simulink model "AFC_FFNN_trainscg_15_15_15_15_15_ctr_Nor_July_15"  (R2021a)
settings: Solver=VariableStepAuto  StartTime=0.0  StopTime=10.0  RelTol=1e-3
libraries: neural x82
(part 3 of 3)

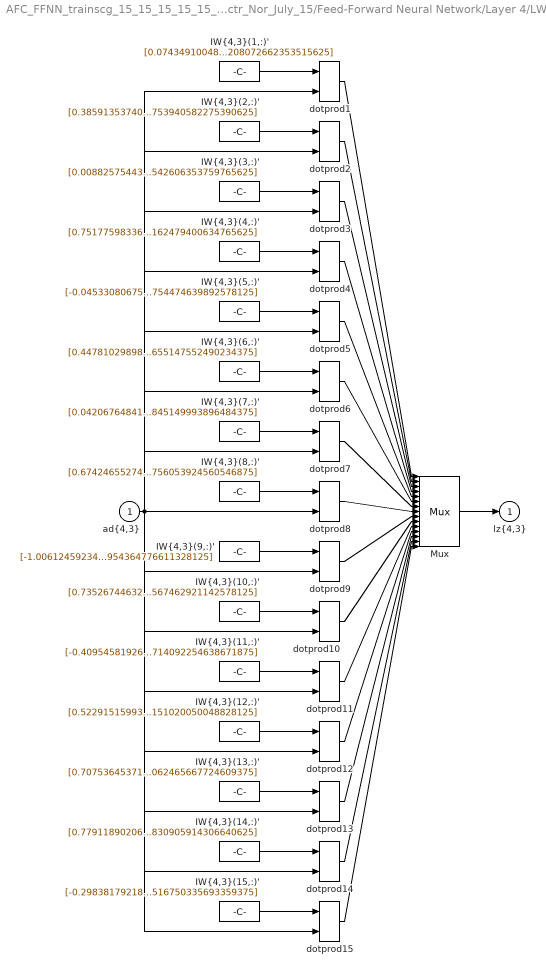
== system AFC_FFNN_trainscg_15_15_15_15_15_ctr_Nor_July_15/Feed-Forward Neural Network/Layer 4/LW{4,3} ==
  "ad{4,3}" : Inport  PortDimensions=15
      mask Display: e = 0.06;c1 = [120 230 180]/255;c2 = ([120 230 180]+0)/(256+128);c3 = ([120 230 180]+128)/(256+128);patch([0 1 1 0],[0 0 1 1],c1);patch([0 1 1 1-e 1-e 0+e],[0 0 1 1-e 0+e 0+e],c2);patch([0 0 1 1-e 0+e 0+e],[0 1 1 1-e 1-e 0+e],c3);plot([0 1 1 0 0],[0 0 1 1 0]);
  "IW{4,3}(1,:)'" : Constant  Value=[0.074349100483344032763710629296838305890560150146484375;-0.2325662791511675653310931011219508945941925048828125;-0.5381154884542291849669481962337158620357513427734375;0.1386295109502034550441607052562176249921321868896484375;-0.37797625642184240479792833866667933762073516845703125;0.6500953139118197388057751595624722540378570556640625;-0.71645051950191429579462010224233381450176239013671875;-0.42415904949149141334174828443792648613452911376953125;-0.522087717682781171646411166875623166561126708984375;0.2134427609428042327266439315280877053737640380859375;-0.9265960947882854181756329126073978841304779052734375;-0.1461549422446244417272964710718952119350433349609375;0.496156728707464911298785636972752399742603302001953125;-0.467980089049811087686947530528414063155651092529296875;-0.828161988219234590502537685097195208072662353515625]
      mask Display: e = 0.06;c1 = [120 150 230]/255;c2 = ([120 150 230]+0)/383;c3 = ([120 150 230]+128)/383;patch([0 1 1 0],[0 0 1 1],c1);patch([0 1 1 1-e 1-e 0+e],[0 0 1 1-e 0+e 0+e],c2);patch([0 0 1 1-e 0+e 0+e],[0 1 1 1-e 1-e 0+e],c3);plot([0 1 1 0 0],[0 0 1 1 0]);disp('weights');
  "IW{4,3}(10,:)'" : Constant  Value=[0.7352674463222312883914355552406050264835357666015625;-0.6220688627615544863402874398161657154560089111328125;-0.4612868378094046040160947086405940353870391845703125;-0.7690744341636996939115533677977509796619415283203125;0.364523315808154446671096593490801751613616943359375;-0.5505544008294369628941922201192937791347503662109375;0.9440421013235733571633545579970814287662506103515625;-0.2344205461328694450884313482674770057201385498046875;-0.3421493061719094175288091719266958534717559814453125;-0.7250516891389173768089904115186072885990142822265625;-0.2911601662961176284483144627301953732967376708984375;0.4865548552326515174826226939330808818340301513671875;-0.614256005760669854254274468985386192798614501953125;-0.14911166211352355759345300612039864063262939453125;0.9353193529802219519098116506938822567462921142578125]
      mask Display: e = 0.06;c1 = [120 150 230]/255;c2 = ([120 150 230]+0)/383;c3 = ([120 150 230]+128)/383;patch([0 1 1 0],[0 0 1 1],c1);patch([0 1 1 1-e 1-e 0+e],[0 0 1 1-e 0+e 0+e],c2);patch([0 0 1 1-e 0+e 0+e],[0 1 1 1-e 1-e 0+e],c3);plot([0 1 1 0 0],[0 0 1 1 0]);disp('weights');
  "IW{4,3}(11,:)'" : Constant  Value=[-0.40954581926718258699793295818381011486053466796875;-0.209952151050021740275042247958481311798095703125;-0.2064904433647580805910592971486039459705352783203125;0.1238876984131753733464620381710119545459747314453125;0.2207973745056917014295549961389042437076568603515625;0.4043229885403072376703903501038439571857452392578125;0.16052297693793082800084448535926640033721923828125;-0.1510627772562316284421513046254403889179229736328125;0.625340446388026105495328010874800384044647216796875;-0.737940333490474387190261040814220905303955078125;-0.081506414055812381747045947122387588024139404296875;0.5640702366617400542736504576168954372406005859375;-0.1445523819865301984322059070109389722347259521484375;-0.573360915257262515609681940986774861812591552734375;0.36503182909853659765531119774095714092254638671875]
      mask Display: e = 0.06;c1 = [120 150 230]/255;c2 = ([120 150 230]+0)/383;c3 = ([120 150 230]+128)/383;patch([0 1 1 0],[0 0 1 1],c1);patch([0 1 1 1-e 1-e 0+e],[0 0 1 1-e 0+e 0+e],c2);patch([0 0 1 1-e 0+e 0+e],[0 1 1 1-e 1-e 0+e],c3);plot([0 1 1 0 0],[0 0 1 1 0]);disp('weights');
  "IW{4,3}(12,:)'" : Constant  Value=[0.5229151599398147443054085670155473053455352783203125;0.0668062429593738738020647360826842486858367919921875;0.10388454329580172619262867783618276007473468780517578125;-0.6445508987129973110796754554030485451221466064453125;0.10760557398696679598515402176417410373687744140625;-0.8975738027855137968202825504704378545284271240234375;0.4048106195281306884936611822922714054584503173828125;0.7646290355386236026191681958152912557125091552734375;0.808722577754244387193693910376168787479400634765625;-0.369588474634115815575796659686602652072906494140625;0.927177911226604312133758867275901138782501220703125;0.2464285148358735799689611667417921125888824462890625;-0.7710168032929891612781148069188930094242095947265625;0.9789119736813682859377649947418831288814544677734375;-0.4766114794815010657913489922066219151020050048828125]
      mask Display: e = 0.06;c1 = [120 150 230]/255;c2 = ([120 150 230]+0)/383;c3 = ([120 150 230]+128)/383;patch([0 1 1 0],[0 0 1 1],c1);patch([0 1 1 1-e 1-e 0+e],[0 0 1 1-e 0+e 0+e],c2);patch([0 0 1 1-e 0+e 0+e],[0 1 1 1-e 1-e 0+e],c3);plot([0 1 1 0 0],[0 0 1 1 0]);disp('weights');
  "IW{4,3}(13,:)'" : Constant  Value=[0.7075364537119337438042521171155385673046112060546875;-0.767668879818697913464120574644766747951507568359375;0.55007147010354884297811395299504511058330535888671875;-0.6106701140328276711244370744680054485797882080078125;0.6972476042524231587549365940503776073455810546875;-0.5354868194475292941802990753785707056522369384765625;0.76167148072680157522285071536316536366939544677734375;-0.42180889329320836456105325851240195333957672119140625;0.7665122361950833518307035774341784417629241943359375;0.90348869713702295580759482618304900825023651123046875;-0.07351895802781971411832273588515818119049072265625;-0.32664730128458874247598942019976675510406494140625;0.6420791870935589340518845347105525434017181396484375;0.74761179512886855036413180641829967498779296875;0.0630118524273972635540985720581375062465667724609375]
      mask Display: e = 0.06;c1 = [120 150 230]/255;c2 = ([120 150 230]+0)/383;c3 = ([120 150 230]+128)/383;patch([0 1 1 0],[0 0 1 1],c1);patch([0 1 1 1-e 1-e 0+e],[0 0 1 1-e 0+e 0+e],c2);patch([0 0 1 1-e 0+e 0+e],[0 1 1 1-e 1-e 0+e],c3);plot([0 1 1 0 0],[0 0 1 1 0]);disp('weights');
  "IW{4,3}(14,:)'" : Constant  Value=[0.77911890206766043487363049280247651040554046630859375;0.3005314436787875909118383788154460489749908447265625;-0.54636206669537357161203772193402983248233795166015625;0.9024541534967465139516207273118197917938232421875;-0.4392096744089373228092654244392178952693939208984375;0.8217256204724023849195191360195167362689971923828125;-0.85371688118925115329460595603450201451778411865234375;0.9714487780644256442741379942162893712520599365234375;-0.324928767306938315329034594469703733921051025390625;-0.18058611694917792167558445726172067224979400634765625;-0.49537725304021062999737523568910546600818634033203125;0.263288327783642639445815802901051938533782958984375;-0.78974407950721126070448008249513804912567138671875;-0.1353463946125611216952933091306476853787899017333984375;-0.76662709328578504397455617436207830905914306640625]
      mask Display: e = 0.06;c1 = [120 150 230]/255;c2 = ([120 150 230]+0)/383;c3 = ([120 150 230]+128)/383;patch([0 1 1 0],[0 0 1 1],c1);patch([0 1 1 1-e 1-e 0+e],[0 0 1 1-e 0+e 0+e],c2);patch([0 0 1 1-e 0+e 0+e],[0 1 1 1-e 1-e 0+e],c3);plot([0 1 1 0 0],[0 0 1 1 0]);disp('weights');
  "IW{4,3}(15,:)'" : Constant  Value=[-0.29838179218397942182861015680828131735324859619140625;-0.37980098378279070203689116169698536396026611328125;-0.713707971537280716489703991101123392581939697265625;0.64570511445325584620746894870535470545291900634765625;0.66287395927729686473384163036826066672801971435546875;0.7270563419832811735687982945819385349750518798828125;-0.80988272704156150094689792240387760102748870849609375;-0.385462680469129070903733236264088191092014312744140625;0.5320320191253158359501185259432531893253326416015625;-0.83917312760953965966592704717186279594898223876953125;0.475406841289294834762557684371131472289562225341796875;-0.577934513428964624637274027918465435504913330078125;0.75053184919748339165579409382189624011516571044921875;-0.38820027172205839871566013243864290416240692138671875;0.5454486372483839939917515948764048516750335693359375]
      mask Display: e = 0.06;c1 = [120 150 230]/255;c2 = ([120 150 230]+0)/383;c3 = ([120 150 230]+128)/383;patch([0 1 1 0],[0 0 1 1],c1);patch([0 1 1 1-e 1-e 0+e],[0 0 1 1-e 0+e 0+e],c2);patch([0 0 1 1-e 0+e 0+e],[0 1 1 1-e 1-e 0+e],c3);plot([0 1 1 0 0],[0 0 1 1 0]);disp('weights');
  "IW{4,3}(2,:)'" : Constant  Value=[0.3859135374030469023409750661812722682952880859375;-0.4894480863430576977890495982137508690357208251953125;-0.8142243049217905426218067077570594847202301025390625;0.26351365588004604934013741512899287045001983642578125;-0.4254725573061353127712891364353708922863006591796875;0.4245532726916321220045347217819653451442718505859375;-0.53889807056561778164649467726121656596660614013671875;-0.86653218037656942751567612504004500806331634521484375;-0.9077254461771564475469631361193023622035980224609375;-0.2742643448700714525756438888492994010448455810546875;0.9801391081252024406467171502299606800079345703125;0.4004532154034503577122450224123895168304443359375;-0.515123397728948884122246454353444278240203857421875;0.83948484916209864525882267116685397922992706298828125;-0.2404448709700057751348367673926986753940582275390625]
      mask Display: e = 0.06;c1 = [120 150 230]/255;c2 = ([120 150 230]+0)/383;c3 = ([120 150 230]+128)/383;patch([0 1 1 0],[0 0 1 1],c1);patch([0 1 1 1-e 1-e 0+e],[0 0 1 1-e 0+e 0+e],c2);patch([0 0 1 1-e 0+e 0+e],[0 1 1 1-e 1-e 0+e],c3);plot([0 1 1 0 0],[0 0 1 1 0]);disp('weights');
  "IW{4,3}(3,:)'" : Constant  Value=[0.00882575443026384874600775987119050114415585994720458984375;-0.062257512940821602143159907427616417407989501953125;0.22176632576290800091811661332030780613422393798828125;0.98680076580737752234284698715782724320888519287109375;0.548050180662683406040969202877022325992584228515625;0.055703066312880356036885132198221981525421142578125;-0.17648508211840396864289459699648432433605194091796875;-0.6791773543076959906983347536879591643810272216796875;0.4688111691864531582751851601642556488513946533203125;0.769869284454610891543779871426522731781005859375;-0.0161893332077034900196021993679096340201795101165771484375;0.6909627908365791881806217133998870849609375;-0.83942374213210302347221158925094641745090484619140625;-0.447167619543548777727437482099048793315887451171875;0.25712671417844124022167306975461542606353759765625]
      mask Display: e = 0.06;c1 = [120 150 230]/255;c2 = ([120 150 230]+0)/383;c3 = ([120 150 230]+128)/383;patch([0 1 1 0],[0 0 1 1],c1);patch([0 1 1 1-e 1-e 0+e],[0 0 1 1-e 0+e 0+e],c2);patch([0 0 1 1-e 0+e 0+e],[0 1 1 1-e 1-e 0+e],c3);plot([0 1 1 0 0],[0 0 1 1 0]);disp('weights');
  "IW{4,3}(4,:)'" : Constant  Value=[0.75177598336575979232065947144292294979095458984375;0.3702895784867925588201842401758767664432525634765625;0.8695032651792422573322483003721572458744049072265625;-0.73114286494634683766236094015766866505146026611328125;-0.821469165834722847563398318015970289707183837890625;-0.860110086194837197837159692426212131977081298828125;-0.98228400009632166334228031701059080660343170166015625;0.17978824004549542880937451627687551081180572509765625;0.619843911574649464313324642716906964778900146484375;0.2170230000325425734342132955134729854762554168701171875;0.5392351431665025618400477469549514353275299072265625;-0.6687457292709984013612256603664718568325042724609375;0.59422170211557101549004755725036375224590301513671875;-0.70772343920246283399677622583112679421901702880859375;-0.15785270237549386962427888647653162479400634765625]
      mask Display: e = 0.06;c1 = [120 150 230]/255;c2 = ([120 150 230]+0)/383;c3 = ([120 150 230]+128)/383;patch([0 1 1 0],[0 0 1 1],c1);patch([0 1 1 1-e 1-e 0+e],[0 0 1 1-e 0+e 0+e],c2);patch([0 0 1 1-e 0+e 0+e],[0 1 1 1-e 1-e 0+e],c3);plot([0 1 1 0 0],[0 0 1 1 0]);disp('weights');
  "IW{4,3}(5,:)'" : Constant  Value=[-0.0453308067579560880488998009241186082363128662109375;-0.360452489509979212556345373741351068019866943359375;-0.908340968616638377852723351679742336273193359375;0.4455634035465834141831464876304380595684051513671875;-0.543489712917239131684254971332848072052001953125;-0.7003784462962896473214868819923140108585357666015625;-0.3159000630638961748530846307403407990932464599609375;-0.731838328583773733981843179208226501941680908203125;-0.194505218857061290549381737946532666683197021484375;-0.8204981840788028168987011667923070490360260009765625;0.017976674577256712694861562340520322322845458984375;-0.7393429432134492884642895660363137722015380859375;-0.8947192019853116295990957951289601624011993408203125;-0.502834162304892640094067246536724269390106201171875;-0.0919987924902649911729213272337801754474639892578125]
      mask Display: e = 0.06;c1 = [120 150 230]/255;c2 = ([120 150 230]+0)/383;c3 = ([120 150 230]+128)/383;patch([0 1 1 0],[0 0 1 1],c1);patch([0 1 1 1-e 1-e 0+e],[0 0 1 1-e 0+e 0+e],c2);patch([0 0 1 1-e 0+e 0+e],[0 1 1 1-e 1-e 0+e],c3);plot([0 1 1 0 0],[0 0 1 1 0]);disp('weights');
  "IW{4,3}(6,:)'" : Constant  Value=[0.4478102989897096986027236198424361646175384521484375;-0.791832975254418425237190604093484580516815185546875;-0.27812353995312122378891217522323131561279296875;-0.4752399215035738588852609609602950513362884521484375;0.9418475099537635397695112260407768189907073974609375;0.4676998024269225506799330105422995984554290771484375;-0.683056658237144898038195606204681098461151123046875;0.5205910196036007686615221246029250323772430419921875;-0.8051914277071781089745172721450217068195343017578125;-0.9068754386092916508488315230351872742176055908203125;-0.146768962619944431935437023639678955078125;0.090061692476291366205032318248413503170013427734375;-0.0920349863494422937293393260915763676166534423828125;-0.90089856406488078022221088758669793605804443359375;0.98467304515324283187283072038553655147552490234375]
      mask Display: e = 0.06;c1 = [120 150 230]/255;c2 = ([120 150 230]+0)/383;c3 = ([120 150 230]+128)/383;patch([0 1 1 0],[0 0 1 1],c1);patch([0 1 1 1-e 1-e 0+e],[0 0 1 1-e 0+e 0+e],c2);patch([0 0 1 1-e 0+e 0+e],[0 1 1 1-e 1-e 0+e],c3);plot([0 1 1 0 0],[0 0 1 1 0]);disp('weights');
  "IW{4,3}(7,:)'" : Constant  Value=[0.042067648411856638224204374409964657388627529144287109375;-0.421486373774265121738835659925825893878936767578125;0.343874306823647390984888261300511658191680908203125;0.79461083619435246561124586150981485843658447265625;0.356971966037631094348370197621989063918590545654296875;-0.9032242250105102510104870816576294600963592529296875;-0.7838942367168808544874991639517247676849365234375;-0.450664356120435705133075998674030415713787078857421875;-0.9820753603085534688688085225294344127178192138671875;-0.66608152346287996525830976679571904242038726806640625;0.1910375355868025593064629674699972383677959442138671875;0.55915736478190769531693149474449455738067626953125;0.53949172083467267224676788828219287097454071044921875;-0.81394298977268497718995376999373547732830047607421875;0.4953742466469905902926029739319346845149993896484375]
      mask Display: e = 0.06;c1 = [120 150 230]/255;c2 = ([120 150 230]+0)/383;c3 = ([120 150 230]+128)/383;patch([0 1 1 0],[0 0 1 1],c1);patch([0 1 1 1-e 1-e 0+e],[0 0 1 1-e 0+e 0+e],c2);patch([0 0 1 1-e 0+e 0+e],[0 1 1 1-e 1-e 0+e],c3);plot([0 1 1 0 0],[0 0 1 1 0]);disp('weights');
  "IW{4,3}(8,:)'" : Constant  Value=[0.6742465527460999030751054306165315210819244384765625;-0.899561043625946243906810195767320692539215087890625;-0.78701267863605373076296700673992745578289031982421875;0.769883275579368753227527122362516820430755615234375;-0.67511918761967637525600594017305411398410797119140625;0.724313351342086964024247208726592361927032470703125;-0.6547149468694486440512037006556056439876556396484375;-0.60395776936510336962982137265498749911785125732421875;-0.9805221777048058751091730300686322152614593505859375;-0.303828044108071682050109529882320202887058258056640625;-0.58397388447369491526472984332940541207790374755859375;-0.6918144040871510025425550338695757091045379638671875;-0.56721303386631849452470532924053259193897247314453125;-0.7694745913482907706537616832065396010875701904296875;-0.8864506383956534119050729714217595756053924560546875]
      mask Display: e = 0.06;c1 = [120 150 230]/255;c2 = ([120 150 230]+0)/383;c3 = ([120 150 230]+128)/383;patch([0 1 1 0],[0 0 1 1],c1);patch([0 1 1 1-e 1-e 0+e],[0 0 1 1-e 0+e 0+e],c2);patch([0 0 1 1-e 0+e 0+e],[0 1 1 1-e 1-e 0+e],c3);plot([0 1 1 0 0],[0 0 1 1 0]);disp('weights');
  "IW{4,3}(9,:)'" : Constant  Value=[-1.0061245923459816165035363155766390264034271240234375;-0.6758029107273058055938008692464791238307952880859375;0.57623520196881783395070897313416935503482818603515625;0.1790242759025365282266051281112595461308956146240234375;-0.414272155068949654577181718195788562297821044921875;-0.015310692783815138540148836909793317317962646484375;0.40768868235542032874008100407081656157970428466796875;-0.73169230261350792776653406690456904470920562744140625;-0.494754223084045374747574896900914609432220458984375;0.51022108874891325402955999379628337919712066650390625;-0.3487405101885940883477132956613786518573760986328125;-0.7242981496196378987662001236458308994770050048828125;0.1746445515014139193699094221301493234932422637939453125;-0.11752990942164535936864666609835694544017314910888671875;-0.0952112383005527807000589746166951954364776611328125]
      mask Display: e = 0.06;c1 = [120 150 230]/255;c2 = ([120 150 230]+0)/383;c3 = ([120 150 230]+128)/383;patch([0 1 1 0],[0 0 1 1],c1);patch([0 1 1 1-e 1-e 0+e],[0 0 1 1-e 0+e 0+e],c2);patch([0 0 1 1-e 0+e 0+e],[0 1 1 1-e 1-e 0+e],c3);plot([0 1 1 0 0],[0 0 1 1 0]);disp('weights');
  Mux : Mux  Inputs=15
      mask Display: e = 0.06;c1 = [120 150 230]/255;c2 = ([120 150 230]+0)/383;c3 = ([120 150 230]+128)/383;patch([0 1 1 0],[0 0 1 1],c1);patch([0 1 1 1-e 1-e 0+e],[0 0 1 1-e 0+e 0+e],c2);patch([0 0 1 1-e 0+e 0+e],[0 1 1 1-e 1-e 0+e],c3);plot([0 1 1 0 0],[0 0 1 1 0]);disp('Mux');
  dotprod{1..15} (15 alike) : neural/Weight Functions/dotprod
  "lz{4,3}" : Outport
      mask Display: e = 0.06;c1 = [120 230 180]/255;c2 = ([120 230 180]+0)/(256+128);c3 = ([120 230 180]+128)/(256+128);patch([0 1 1 0],[0 0 1 1],c1);patch([0 1 1 1-e 1-e 0+e],[0 0 1 1-e 0+e 0+e],c2);patch([0 0 1 1-e 0+e 0+e],[0 1 1 1-e 1-e 0+e],c3);plot([0 1 1 0 0],[0 0 1 1 0]);
  wires:
  "IW{4,3}(1,:)'"/1 -> dotprod1/1
  "ad{4,3}"/1 -> dotprod1/2, dotprod2/2, dotprod3/2, dotprod4/2, dotprod5/2, dotprod6/2, dotprod7/2, dotprod8/2, dotprod9/2, dotprod10/2, dotprod11/2, dotprod12/2, dotprod13/2, dotprod14/2, dotprod15/2
  dotprod1/1 -> Mux/1
  "IW{4,3}(2,:)'"/1 -> dotprod2/1
  dotprod2/1 -> Mux/2
  "IW{4,3}(3,:)'"/1 -> dotprod3/1
  dotprod3/1 -> Mux/3
  "IW{4,3}(4,:)'"/1 -> dotprod4/1
  dotprod4/1 -> Mux/4
  "IW{4,3}(5,:)'"/1 -> dotprod5/1
  dotprod5/1 -> Mux/5
  "IW{4,3}(6,:)'"/1 -> dotprod6/1
  dotprod6/1 -> Mux/6
  "IW{4,3}(7,:)'"/1 -> dotprod7/1
  dotprod7/1 -> Mux/7
  "IW{4,3}(8,:)'"/1 -> dotprod8/1
  dotprod8/1 -> Mux/8
  "IW{4,3}(9,:)'"/1 -> dotprod9/1
  dotprod9/1 -> Mux/9
  "IW{4,3}(10,:)'"/1 -> dotprod10/1
  dotprod10/1 -> Mux/10
  "IW{4,3}(11,:)'"/1 -> dotprod11/1
  dotprod11/1 -> Mux/11
  "IW{4,3}(12,:)'"/1 -> dotprod12/1
  dotprod12/1 -> Mux/12
  "IW{4,3}(13,:)'"/1 -> dotprod13/1
  dotprod13/1 -> Mux/13
  "IW{4,3}(14,:)'"/1 -> dotprod14/1
  dotprod14/1 -> Mux/14
  "IW{4,3}(15,:)'"/1 -> dotprod15/1
  dotprod15/1 -> Mux/15
  Mux/1 -> "lz{4,3}"/1

== system AFC_FFNN_trainscg_15_15_15_15_15_ctr_Nor_July_15/Feed-Forward Neural Network/Layer 5/Delays 1 ==
  "p{5}" : Inport  PortDimensions=15
      mask Display: e = 0.06;c1 = [120 230 180]/255;c2 = ([120 230 180]+0)/(256+128);c3 = ([120 230 180]+128)/(256+128);patch([0 1 1 0],[0 0 1 1],c1);patch([0 1 1 1-e 1-e 0+e],[0 0 1 1-e 0+e 0+e],c2);patch([0 0 1 1-e 0+e 0+e],[0 1 1 1-e 1-e 0+e],c3);plot([0 1 1 0 0],[0 0 1 1 0]);
  mux : Mux  Inputs=1
      mask Display: e = 0.06;c1 = [120 150 230]/255;c2 = ([120 150 230]+0)/383;c3 = ([120 150 230]+128)/383;patch([0 1 1 0],[0 0 1 1],c1);patch([0 1 1 1-e 1-e 0+e],[0 0 1 1-e 0+e 0+e],c2);patch([0 0 1 1-e 0+e 0+e],[0 1 1 1-e 1-e 0+e],c3);plot([0 1 1 0 0],[0 0 1 1 0]);disp('Mux')
  "pd{5,4}" : Outport
      mask Display: e = 0.06;c1 = [120 230 180]/255;c2 = ([120 230 180]+0)/(256+128);c3 = ([120 230 180]+128)/(256+128);patch([0 1 1 0],[0 0 1 1],c1);patch([0 1 1 1-e 1-e 0+e],[0 0 1 1-e 0+e 0+e],c2);patch([0 0 1 1-e 0+e 0+e],[0 1 1 1-e 1-e 0+e],c3);plot([0 1 1 0 0],[0 0 1 1 0]);
  wires:
  "p{5}"/1 -> mux/1
  mux/1 -> "pd{5,4}"/1

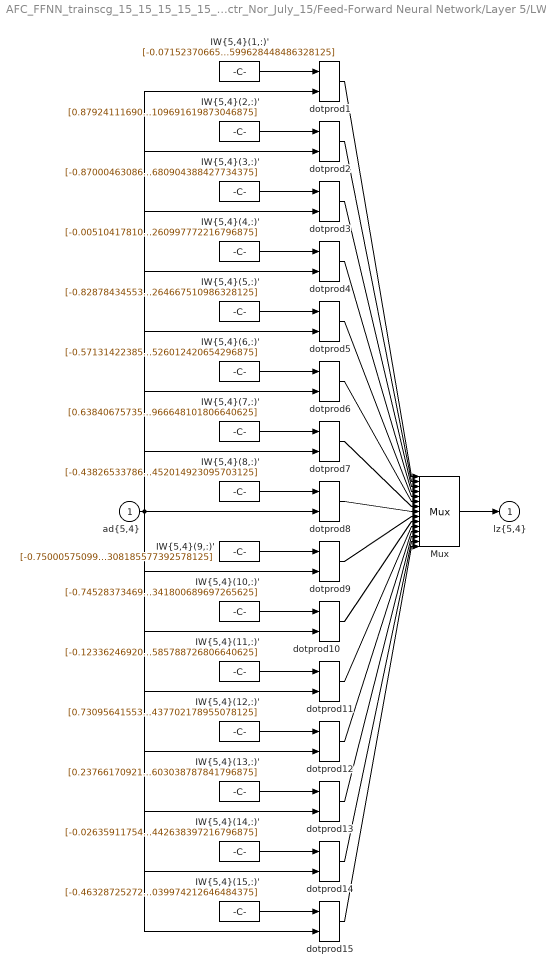
== system AFC_FFNN_trainscg_15_15_15_15_15_ctr_Nor_July_15/Feed-Forward Neural Network/Layer 5/LW{5,4} ==
  "ad{5,4}" : Inport  PortDimensions=15
      mask Display: e = 0.06;c1 = [120 230 180]/255;c2 = ([120 230 180]+0)/(256+128);c3 = ([120 230 180]+128)/(256+128);patch([0 1 1 0],[0 0 1 1],c1);patch([0 1 1 1-e 1-e 0+e],[0 0 1 1-e 0+e 0+e],c2);patch([0 0 1 1-e 0+e 0+e],[0 1 1 1-e 1-e 0+e],c3);plot([0 1 1 0 0],[0 0 1 1 0]);
  "IW{5,4}(1,:)'" : Constant  Value=[-0.0715237066501865637047075097143533639609813690185546875;-0.059455360452374352020488146308707655407488346099853515625;0.0042080898735644862995730619559253682382404804229736328125;0.2901089383986412695293211072566919028759002685546875;0.095073068854255371462613766198046505451202392578125;-0.7245204898788843994594799369224347174167633056640625;-0.95341156977462160337921659447601996362209320068359375;-0.381546919757219826774274906711070798337459564208984375;0.64062838445033254419769264131900854408740997314453125;-0.41532270884854227688265382312238216400146484375;0.9228342233845399089631200695293955504894256591796875;0.52678841002817666794300066612777300179004669189453125;0.92917047870120661468007483563269488513469696044921875;0.31486675897001215052029010621481575071811676025390625;0.0978604704135155600841500245223869569599628448486328125]
      mask Display: e = 0.06;c1 = [120 150 230]/255;c2 = ([120 150 230]+0)/383;c3 = ([120 150 230]+128)/383;patch([0 1 1 0],[0 0 1 1],c1);patch([0 1 1 1-e 1-e 0+e],[0 0 1 1-e 0+e 0+e],c2);patch([0 0 1 1-e 0+e 0+e],[0 1 1 1-e 1-e 0+e],c3);plot([0 1 1 0 0],[0 0 1 1 0]);disp('weights');
  "IW{5,4}(10,:)'" : Constant  Value=[-0.745283734691431387631155303097330033779144287109375;0.6327139929387517458536649428424425423145294189453125;0.1814176919217727335098544472202775068581104278564453125;0.44811074278119722436031224788166582584381103515625;-0.8904745653823924467218375866650603711605072021484375;-0.1411457300286087512830590640078298747539520263671875;0.6893492671787264658433969088946469128131866455078125;-0.92286808214381721438002159629832021892070770263671875;-0.702719569569371316219985601492226123809814453125;0.578347130669404574376812888658605515956878662109375;-0.433450867120990235292765646590851247310638427734375;-0.10595183853206820157044631969256442971527576446533203125;0.05814803339909381529881926553571247495710849761962890625;0.70409350150412330915372649542405270040035247802734375;0.49499370589664215547287540175602771341800689697265625]
      mask Display: e = 0.06;c1 = [120 150 230]/255;c2 = ([120 150 230]+0)/383;c3 = ([120 150 230]+128)/383;patch([0 1 1 0],[0 0 1 1],c1);patch([0 1 1 1-e 1-e 0+e],[0 0 1 1-e 0+e 0+e],c2);patch([0 0 1 1-e 0+e 0+e],[0 1 1 1-e 1-e 0+e],c3);plot([0 1 1 0 0],[0 0 1 1 0]);disp('weights');
  "IW{5,4}(11,:)'" : Constant  Value=[-0.1233624692016876689404369926705840043723583221435546875;0.7427858565377867261503297413582913577556610107421875;-0.6452270479684789616925399968749843537807464599609375;0.80229201087052237628682860304252244532108306884765625;-0.0568868193236429231518513915943913161754608154296875;0.6812541647223564478252910703304223716259002685546875;0.73478538636070300782421327312476933002471923828125;-0.90683981762392529279992459123604930937290191650390625;0.1533706191209432689870340027482598088681697845458984375;-0.2065977000624570347753206078778021037578582763671875;-0.69917607959227812131075552315451204776763916015625;0.26674758647147456258608144707977771759033203125;0.00914836505551542243652729524683309136889874935150146484375;-0.6399491125429499494003948711906559765338897705078125;0.0354412162674015152052930943682440556585788726806640625]
      mask Display: e = 0.06;c1 = [120 150 230]/255;c2 = ([120 150 230]+0)/383;c3 = ([120 150 230]+128)/383;patch([0 1 1 0],[0 0 1 1],c1);patch([0 1 1 1-e 1-e 0+e],[0 0 1 1-e 0+e 0+e],c2);patch([0 0 1 1-e 0+e 0+e],[0 1 1 1-e 1-e 0+e],c3);plot([0 1 1 0 0],[0 0 1 1 0]);disp('weights');
  "IW{5,4}(12,:)'" : Constant  Value=[0.73095641553966250736351639716303907334804534912109375;0.4871355339961243036128735184320248663425445556640625;-0.497421269660421050406995391313103027641773223876953125;0.797168206723321670637005809112451970577239990234375;0.417766150048340278999603469856083393096923828125;0.6564646990516640467916431589401327073574066162109375;0.7871861509157020986293673558975569903850555419921875;0.19888839208758846144320386883919127285480499267578125;0.83553010432982921518174634911702014505863189697265625;-0.411943496993746993695140190538950264453887939453125;0.922024497362436523673068222706206142902374267578125;0.518401102529268964502762173651717603206634521484375;-0.87560721497756077713603417578269727528095245361328125;0.57175513701463687166182126020430587232112884521484375;-0.8276073568365678312375166569836437702178955078125]
      mask Display: e = 0.06;c1 = [120 150 230]/255;c2 = ([120 150 230]+0)/383;c3 = ([120 150 230]+128)/383;patch([0 1 1 0],[0 0 1 1],c1);patch([0 1 1 1-e 1-e 0+e],[0 0 1 1-e 0+e 0+e],c2);patch([0 0 1 1-e 0+e 0+e],[0 1 1 1-e 1-e 0+e],c3);plot([0 1 1 0 0],[0 0 1 1 0]);disp('weights');
  "IW{5,4}(13,:)'" : Constant  Value=[0.2376617092170787426397282615653239190578460693359375;-0.9885705088057334943840714913676492869853973388671875;-0.886880268826178763674761285074055194854736328125;0.7061210321519670873868790295091457664966583251953125;-0.6273662474377628139876605928293429315090179443359375;-0.998268267412152798812030596309341490268707275390625;-0.4703689472235585977699656723416410386562347412109375;-0.9241992366964633109915894237929023802280426025390625;-0.747719904959309733527561547816731035709381103515625;0.8818924664208236396945039814454503357410430908203125;0.07674704745712279674307865207083523273468017578125;-0.4112203622036787464821827597916126251220703125;0.83385659205751228029157573473639786243438720703125;-0.25162142736245396434924259665422141551971435546875;-0.180344219235205827089885133318603038787841796875]
      mask Display: e = 0.06;c1 = [120 150 230]/255;c2 = ([120 150 230]+0)/383;c3 = ([120 150 230]+128)/383;patch([0 1 1 0],[0 0 1 1],c1);patch([0 1 1 1-e 1-e 0+e],[0 0 1 1-e 0+e 0+e],c2);patch([0 0 1 1-e 0+e 0+e],[0 1 1 1-e 1-e 0+e],c3);plot([0 1 1 0 0],[0 0 1 1 0]);disp('weights');
  "IW{5,4}(14,:)'" : Constant  Value=[-0.0263591175497553918682935858441851451061666011810302734375;-0.73862473877419976275859880843199789524078369140625;-0.9818407470620658106241762652643956243991851806640625;-0.8322907510546138087903500490938313305377960205078125;-0.40775753473065368126526664127595722675323486328125;0.85727737303545215041822302737273275852203369140625;-0.913714783630615645648731515393592417240142822265625;-0.434025787294483100797748420518473722040653228759765625;0.51057369949210862358768281410448253154754638671875;-0.923275801188926603657591840601526200771331787109375;-0.6364652652927833553775371910887770354747772216796875;0.7604639939080046762143183514126576483249664306640625;0.559391998498745213197480552480556070804595947265625;0.51465198508545284550308451798628084361553192138671875;0.40409177873949164716549375953036360442638397216796875]
      mask Display: e = 0.06;c1 = [120 150 230]/255;c2 = ([120 150 230]+0)/383;c3 = ([120 150 230]+128)/383;patch([0 1 1 0],[0 0 1 1],c1);patch([0 1 1 1-e 1-e 0+e],[0 0 1 1-e 0+e 0+e],c2);patch([0 0 1 1-e 0+e 0+e],[0 1 1 1-e 1-e 0+e],c3);plot([0 1 1 0 0],[0 0 1 1 0]);disp('weights');
  "IW{5,4}(15,:)'" : Constant  Value=[-0.46328725272275139701605439768172800540924072265625;-0.141458750541851419058048122678883373737335205078125;0.417359177593134678119213276659138500690460205078125;-0.7778940511957792569575076413457281887531280517578125;-0.274320322427507701235072090639732778072357177734375;-0.7019314613676590486335271634743548929691314697265625;-0.7879876969556496302260484299040399491786956787109375;0.7965061683491236887988407033844850957393646240234375;0.2892567451407488388070987639366649091243743896484375;-0.805571707848603768553630288806743919849395751953125;-0.163626497462990183606734717614017426967620849609375;-0.683466400463462964154359724489040672779083251953125;-0.2210723476022076194880128241493366658687591552734375;-0.8756542550710353367549032554961740970611572265625;-0.0916336575431715427697554332553409039974212646484375]
      mask Display: e = 0.06;c1 = [120 150 230]/255;c2 = ([120 150 230]+0)/383;c3 = ([120 150 230]+128)/383;patch([0 1 1 0],[0 0 1 1],c1);patch([0 1 1 1-e 1-e 0+e],[0 0 1 1-e 0+e 0+e],c2);patch([0 0 1 1-e 0+e 0+e],[0 1 1 1-e 1-e 0+e],c3);plot([0 1 1 0 0],[0 0 1 1 0]);disp('weights');
  "IW{5,4}(2,:)'" : Constant  Value=[0.8792411169036473683746635288116522133350372314453125;0.9476643750844193636595491625485010445117950439453125;-0.121014662404281547747331160280737094581127166748046875;-0.64955468710774566520882444820017553865909576416015625;-0.2192888029702277918886466068215668201446533203125;0.9482089460418883231085374063695780932903289794921875;0.81071456577514011687668471495271660387516021728515625;-0.8778539344975506697466016703401692211627960205078125;-0.5367666595045050836887412515352480113506317138671875;-0.0818759946323519560706927222781814634799957275390625;-0.00147913782462527620964465313591063022613525390625;0.97707803825832273414420114931999705731868743896484375;-0.57967360625535724327761499807820655405521392822265625;0.7041045664752501043182064677239395678043365478515625;-0.71981214912070068390193000595900230109691619873046875]
      mask Display: e = 0.06;c1 = [120 150 230]/255;c2 = ([120 150 230]+0)/383;c3 = ([120 150 230]+128)/383;patch([0 1 1 0],[0 0 1 1],c1);patch([0 1 1 1-e 1-e 0+e],[0 0 1 1-e 0+e 0+e],c2);patch([0 0 1 1-e 0+e 0+e],[0 1 1 1-e 1-e 0+e],c3);plot([0 1 1 0 0],[0 0 1 1 0]);disp('weights');
  "IW{5,4}(3,:)'" : Constant  Value=[-0.870004630865640837811270102974958717823028564453125;-0.1394130191014479880351473184418864548206329345703125;0.44929842102961747851708196321851573884487152099609375;0.9390056072431598455096946054254658520221710205078125;0.3392077142091143304725164853152818977832794189453125;0.2638263459878500416522228988469578325748443603515625;-0.1271702216377524063961601541450363583862781524658203125;0.824871971464007369689852566807530820369720458984375;0.752978288612214274877487696358002722263336181640625;-0.358871719956378232296856367611326277256011962890625;0.3877730536909573810788742775912396609783172607421875;-0.1622420881467621089910835507907904684543609619140625;0.23014593691751572546166926258592866361141204833984375;-0.88941897035361938694819627926335670053958892822265625;-0.74207495222659980438351112752570770680904388427734375]
      mask Display: e = 0.06;c1 = [120 150 230]/255;c2 = ([120 150 230]+0)/383;c3 = ([120 150 230]+128)/383;patch([0 1 1 0],[0 0 1 1],c1);patch([0 1 1 1-e 1-e 0+e],[0 0 1 1-e 0+e 0+e],c2);patch([0 0 1 1-e 0+e 0+e],[0 1 1 1-e 1-e 0+e],c3);plot([0 1 1 0 0],[0 0 1 1 0]);disp('weights');
  "IW{5,4}(4,:)'" : Constant  Value=[-0.005104178107196749754337350424293617834337055683135986328125;0.723242918597417627779577742330729961395263671875;0.1777800728242972805315247342150541953742504119873046875;-0.2315142766680377828247827665109070949256420135498046875;0.66432988641756995917830863618291914463043212890625;-0.4486087512464720372662441150168888270854949951171875;-0.96268451305722180233459539522300474345684051513671875;-0.5291219806882916376622461029910482466220855712890625;-0.6246384153151449680763107608072459697723388671875;-0.7168661734093217940966269452474080026149749755859375;0.163315871632827569470691742026247084140777587890625;-0.6104447643185764160733697281102649867534637451171875;0.58602976789892957665273343081935308873653411865234375;0.88462651353997456826760981130064465105533599853515625;0.2406072415787565699218930603819899260997772216796875]
      mask Display: e = 0.06;c1 = [120 150 230]/255;c2 = ([120 150 230]+0)/383;c3 = ([120 150 230]+128)/383;patch([0 1 1 0],[0 0 1 1],c1);patch([0 1 1 1-e 1-e 0+e],[0 0 1 1-e 0+e 0+e],c2);patch([0 0 1 1-e 0+e 0+e],[0 1 1 1-e 1-e 0+e],c3);plot([0 1 1 0 0],[0 0 1 1 0]);disp('weights');
  "IW{5,4}(5,:)'" : Constant  Value=[-0.8287843455345054177740848899702541530132293701171875;0.60702538017370255563065484238904900848865509033203125;-0.19355408020178421768520138357416726648807525634765625;0.8884086963255166669028994874679483473300933837890625;0.02810771528634337101948403869755566120147705078125;-0.05301070772614746573481170344166457653045654296875;-0.65137729229106067219134956758352927863597869873046875;0.4202804667444233199802283706958405673503875732421875;-0.57904508252670738865930388783453963696956634521484375;0.5686244136944262894672874608659185469150543212890625;-0.328574866563430934007783434935845434665679931640625;0.0905545868520955254954429847202845849096775054931640625;-0.349451482700606330666914800531230866909027099609375;0.042456016757196547717345680439393618144094944000244140625;0.1761051545277756702478910710851778276264667510986328125]
      mask Display: e = 0.06;c1 = [120 150 230]/255;c2 = ([120 150 230]+0)/383;c3 = ([120 150 230]+128)/383;patch([0 1 1 0],[0 0 1 1],c1);patch([0 1 1 1-e 1-e 0+e],[0 0 1 1-e 0+e 0+e],c2);patch([0 0 1 1-e 0+e 0+e],[0 1 1 1-e 1-e 0+e],c3);plot([0 1 1 0 0],[0 0 1 1 0]);disp('weights');
  "IW{5,4}(6,:)'" : Constant  Value=[-0.5713142238533446271020466156187467277050018310546875;-0.503576738999999662382833776064217090606689453125;-0.6481484936093604432016945793293416500091552734375;-0.1183454483920598765411824615512159653007984161376953125;0.8834983524723070136275282493443228304386138916015625;-0.7475172422529510196653745879302732646465301513671875;-1.0046336664456265719280736448126845061779022216796875;0.608725088947579706655233167111873626708984375;0.499049521527679729171467215564916841685771942138671875;0.52599052748356456277178949676454067230224609375;0.2859724590846799419097123973187990486621856689453125;-0.75506229605684749284222334608784876763820648193359375;-0.384006528183055750869101530042826198041439056396484375;0.59518858313426858952510656308731995522975921630859375;-0.3364401719934875245598959736526012420654296875]
      mask Display: e = 0.06;c1 = [120 150 230]/255;c2 = ([120 150 230]+0)/383;c3 = ([120 150 230]+128)/383;patch([0 1 1 0],[0 0 1 1],c1);patch([0 1 1 1-e 1-e 0+e],[0 0 1 1-e 0+e 0+e],c2);patch([0 0 1 1-e 0+e 0+e],[0 1 1 1-e 1-e 0+e],c3);plot([0 1 1 0 0],[0 0 1 1 0]);disp('weights');
  "IW{5,4}(7,:)'" : Constant  Value=[0.6384067573591323263570984636317007243633270263671875;-0.398906189376702524640450064907781779766082763671875;0.3590663490432792759321500852820463478565216064453125;0.9824522582283503613354014305514283478260040283203125;-0.1817236106276645113410950216348282992839813232421875;0.33684980648238660450033421511761844158172607421875;-0.63399701385133511166714015416800975799560546875;-0.7621407404871585189454208375536836683750152587890625;-0.8769903337800799558721109860925935208797454833984375;-0.4675323855823581009616418668883852660655975341796875;-0.805696629997617375096297109848819673061370849609375;-0.4819410402133545989755702976253814995288848876953125;0.496426452433425868804306446691043674945831298828125;-0.51429089900277258351479758857749402523040771484375;-0.3450216144076565516485288753756321966648101806640625]
      mask Display: e = 0.06;c1 = [120 150 230]/255;c2 = ([120 150 230]+0)/383;c3 = ([120 150 230]+128)/383;patch([0 1 1 0],[0 0 1 1],c1);patch([0 1 1 1-e 1-e 0+e],[0 0 1 1-e 0+e 0+e],c2);patch([0 0 1 1-e 0+e 0+e],[0 1 1 1-e 1-e 0+e],c3);plot([0 1 1 0 0],[0 0 1 1 0]);disp('weights');
  "IW{5,4}(8,:)'" : Constant  Value=[-0.43826533786090704492011127513251267373561859130859375;-0.177428161616140556144927131754229776561260223388671875;-0.55432434021778254074064307133085094392299652099609375;0.1574437223343636838013281931125675328075885772705078125;0.4222152666047025437734419028856791555881500244140625;0.669107579605679791967531855334527790546417236328125;-0.89015338475136795981512705111526884138584136962890625;-0.81263781446701732757986746946698985993862152099609375;-0.73447676533593952985512487430241890251636505126953125;-0.881409950336343950283435333403758704662322998046875;0.5306763737125665958416220746585167944431304931640625;-0.258124212915001260970626617563539184629917144775390625;0.60220637617682515330130854636081494390964508056640625;0.59081506636078129357514399089268408715724945068359375;0.5258786458552944242939020114135928452014923095703125]
      mask Display: e = 0.06;c1 = [120 150 230]/255;c2 = ([120 150 230]+0)/383;c3 = ([120 150 230]+128)/383;patch([0 1 1 0],[0 0 1 1],c1);patch([0 1 1 1-e 1-e 0+e],[0 0 1 1-e 0+e 0+e],c2);patch([0 0 1 1-e 0+e 0+e],[0 1 1 1-e 1-e 0+e],c3);plot([0 1 1 0 0],[0 0 1 1 0]);disp('weights');
  "IW{5,4}(9,:)'" : Constant  Value=[-0.75000575099870292472559185625868849456310272216796875;0.79529760800211957150196440125000663101673126220703125;0.6376047718358714977426870973431505262851715087890625;-0.483394652199553409577248430650797672569751739501953125;0.103791975354226462258111496339552104473114013671875;-0.471845248230328362382124396390281617641448974609375;0.394311694379341604044242330928682349622249603271484375;0.26681610727024551721342504606582224369049072265625;0.84738192844972914929968510477920062839984893798828125;0.2339243378057733746544499808805994689464569091796875;0.8609789815849964167426833228091709315776824951171875;0.9634103237621685078551081460318528115749359130859375;0.191715289750559458870071694036596454679965972900390625;-0.29679487907828738801896406585001386702060699462890625;0.8576116780544318363155298357014544308185577392578125]
      mask Display: e = 0.06;c1 = [120 150 230]/255;c2 = ([120 150 230]+0)/383;c3 = ([120 150 230]+128)/383;patch([0 1 1 0],[0 0 1 1],c1);patch([0 1 1 1-e 1-e 0+e],[0 0 1 1-e 0+e 0+e],c2);patch([0 0 1 1-e 0+e 0+e],[0 1 1 1-e 1-e 0+e],c3);plot([0 1 1 0 0],[0 0 1 1 0]);disp('weights');
  Mux : Mux  Inputs=15
      mask Display: e = 0.06;c1 = [120 150 230]/255;c2 = ([120 150 230]+0)/383;c3 = ([120 150 230]+128)/383;patch([0 1 1 0],[0 0 1 1],c1);patch([0 1 1 1-e 1-e 0+e],[0 0 1 1-e 0+e 0+e],c2);patch([0 0 1 1-e 0+e 0+e],[0 1 1 1-e 1-e 0+e],c3);plot([0 1 1 0 0],[0 0 1 1 0]);disp('Mux');
  dotprod{1..15} (15 alike) : neural/Weight Functions/dotprod
  "lz{5,4}" : Outport
      mask Display: e = 0.06;c1 = [120 230 180]/255;c2 = ([120 230 180]+0)/(256+128);c3 = ([120 230 180]+128)/(256+128);patch([0 1 1 0],[0 0 1 1],c1);patch([0 1 1 1-e 1-e 0+e],[0 0 1 1-e 0+e 0+e],c2);patch([0 0 1 1-e 0+e 0+e],[0 1 1 1-e 1-e 0+e],c3);plot([0 1 1 0 0],[0 0 1 1 0]);
  wires:
  "IW{5,4}(1,:)'"/1 -> dotprod1/1
  "ad{5,4}"/1 -> dotprod1/2, dotprod2/2, dotprod3/2, dotprod4/2, dotprod5/2, dotprod6/2, dotprod7/2, dotprod8/2, dotprod9/2, dotprod10/2, dotprod11/2, dotprod12/2, dotprod13/2, dotprod14/2, dotprod15/2
  dotprod1/1 -> Mux/1
  "IW{5,4}(2,:)'"/1 -> dotprod2/1
  dotprod2/1 -> Mux/2
  "IW{5,4}(3,:)'"/1 -> dotprod3/1
  dotprod3/1 -> Mux/3
  "IW{5,4}(4,:)'"/1 -> dotprod4/1
  dotprod4/1 -> Mux/4
  "IW{5,4}(5,:)'"/1 -> dotprod5/1
  dotprod5/1 -> Mux/5
  "IW{5,4}(6,:)'"/1 -> dotprod6/1
  dotprod6/1 -> Mux/6
  "IW{5,4}(7,:)'"/1 -> dotprod7/1
  dotprod7/1 -> Mux/7
  "IW{5,4}(8,:)'"/1 -> dotprod8/1
  dotprod8/1 -> Mux/8
  "IW{5,4}(9,:)'"/1 -> dotprod9/1
  dotprod9/1 -> Mux/9
  "IW{5,4}(10,:)'"/1 -> dotprod10/1
  dotprod10/1 -> Mux/10
  "IW{5,4}(11,:)'"/1 -> dotprod11/1
  dotprod11/1 -> Mux/11
  "IW{5,4}(12,:)'"/1 -> dotprod12/1
  dotprod12/1 -> Mux/12
  "IW{5,4}(13,:)'"/1 -> dotprod13/1
  dotprod13/1 -> Mux/13
  "IW{5,4}(14,:)'"/1 -> dotprod14/1
  dotprod14/1 -> Mux/14
  "IW{5,4}(15,:)'"/1 -> dotprod15/1
  dotprod15/1 -> Mux/15
  Mux/1 -> "lz{5,4}"/1

== system AFC_FFNN_trainscg_15_15_15_15_15_ctr_Nor_July_15/Feed-Forward Neural Network/Layer 6/Delays 1 ==
  "p{6}" : Inport  PortDimensions=15
      mask Display: e = 0.06;c1 = [120 230 180]/255;c2 = ([120 230 180]+0)/(256+128);c3 = ([120 230 180]+128)/(256+128);patch([0 1 1 0],[0 0 1 1],c1);patch([0 1 1 1-e 1-e 0+e],[0 0 1 1-e 0+e 0+e],c2);patch([0 0 1 1-e 0+e 0+e],[0 1 1 1-e 1-e 0+e],c3);plot([0 1 1 0 0],[0 0 1 1 0]);
  mux : Mux  Inputs=1
      mask Display: e = 0.06;c1 = [120 150 230]/255;c2 = ([120 150 230]+0)/383;c3 = ([120 150 230]+128)/383;patch([0 1 1 0],[0 0 1 1],c1);patch([0 1 1 1-e 1-e 0+e],[0 0 1 1-e 0+e 0+e],c2);patch([0 0 1 1-e 0+e 0+e],[0 1 1 1-e 1-e 0+e],c3);plot([0 1 1 0 0],[0 0 1 1 0]);disp('Mux')
  "pd{6,5}" : Outport
      mask Display: e = 0.06;c1 = [120 230 180]/255;c2 = ([120 230 180]+0)/(256+128);c3 = ([120 230 180]+128)/(256+128);patch([0 1 1 0],[0 0 1 1],c1);patch([0 1 1 1-e 1-e 0+e],[0 0 1 1-e 0+e 0+e],c2);patch([0 0 1 1-e 0+e 0+e],[0 1 1 1-e 1-e 0+e],c3);plot([0 1 1 0 0],[0 0 1 1 0]);
  wires:
  "p{6}"/1 -> mux/1
  mux/1 -> "pd{6,5}"/1

== system AFC_FFNN_trainscg_15_15_15_15_15_ctr_Nor_July_15/Feed-Forward Neural Network/Layer 6/LW{6,5} ==
  "ad{6,5}" : Inport  PortDimensions=15
      mask Display: e = 0.06;c1 = [120 230 180]/255;c2 = ([120 230 180]+0)/(256+128);c3 = ([120 230 180]+128)/(256+128);patch([0 1 1 0],[0 0 1 1],c1);patch([0 1 1 1-e 1-e 0+e],[0 0 1 1-e 0+e 0+e],c2);patch([0 0 1 1-e 0+e 0+e],[0 1 1 1-e 1-e 0+e],c3);plot([0 1 1 0 0],[0 0 1 1 0]);
  "IW{6,5}(1,:)'" : Constant  Value=[-0.123794355159188906867484547547064721584320068359375;-0.54342989784435513644922366438549943268299102783203125;0.67191439248000695005913485147175379097461700439453125;-0.52498234414585687179766182453022338449954986572265625;-0.467335260607861291415332516407943330705165863037109375;-0.199615927195639308866503824901883490383625030517578125;0.21435004773181720594266153057105839252471923828125;0.91169194707349332507106964840204454958438873291015625;0.02540510237598773979339483730655047111213207244873046875;0.63533396914472561878284295744379051029682159423828125;-0.1332576588371870152105458373625879175961017608642578125;-0.57005408254605860474129030990297906100749969482421875;-0.0886450937949223582990043723839335143566131591796875;0.36612079421426901859604186029173433780670166015625;-0.1895090319374348464265267466544173657894134521484375]
      mask Display: e = 0.06;c1 = [120 150 230]/255;c2 = ([120 150 230]+0)/383;c3 = ([120 150 230]+128)/383;patch([0 1 1 0],[0 0 1 1],c1);patch([0 1 1 1-e 1-e 0+e],[0 0 1 1-e 0+e 0+e],c2);patch([0 0 1 1-e 0+e 0+e],[0 1 1 1-e 1-e 0+e],c3);plot([0 1 1 0 0],[0 0 1 1 0]);disp('weights');
  Mux : Mux  Inputs=1
      mask Display: e = 0.06;c1 = [120 150 230]/255;c2 = ([120 150 230]+0)/383;c3 = ([120 150 230]+128)/383;patch([0 1 1 0],[0 0 1 1],c1);patch([0 1 1 1-e 1-e 0+e],[0 0 1 1-e 0+e 0+e],c2);patch([0 0 1 1-e 0+e 0+e],[0 1 1 1-e 1-e 0+e],c3);plot([0 1 1 0 0],[0 0 1 1 0]);disp('Mux');
  dotprod1 : neural/Weight Functions/dotprod
  "lz{6,5}" : Outport
      mask Display: e = 0.06;c1 = [120 230 180]/255;c2 = ([120 230 180]+0)/(256+128);c3 = ([120 230 180]+128)/(256+128);patch([0 1 1 0],[0 0 1 1],c1);patch([0 1 1 1-e 1-e 0+e],[0 0 1 1-e 0+e 0+e],c2);patch([0 0 1 1-e 0+e 0+e],[0 1 1 1-e 1-e 0+e],c3);plot([0 1 1 0 0],[0 0 1 1 0]);
  wires:
  "IW{6,5}(1,:)'"/1 -> dotprod1/1
  "ad{6,5}"/1 -> dotprod1/2
  dotprod1/1 -> Mux/1
  Mux/1 -> "lz{6,5}"/1
